simulink library "NxSwcLib"  (R2024a)
settings: Solver=VariableStepAuto  StartTime=0.0  StopTime=10.0  RelTol=1e-3
undefined symbols (not defined in the file or in its folder): QLF_DEBOUNCE, QLF_ERROR_RANGE, QLF_OK
libraries: simulink x4
Description:
  | SPDX-License-Identifier: Apache-2.0. neXtBSW block library for software components (RTE-07), generated by tools/swc/swc_lib_create.m - do not edit by hand.
settings Model: Creator=danie  LastModifiedBy=danie

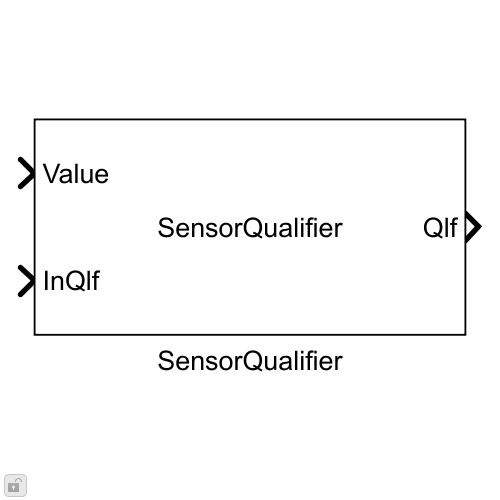
[thumbnail: Simulink's stored preview of the top-level diagram]
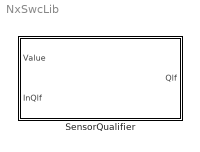
== system NxSwcLib ==
  SensorQualifier : Subsystem  mask(neXtBSW Sensor Qualifier){min_value=0, max_value=4095, debounce_ms=0}
      mask prompts: min_value "Lowest valid value (inclusive, unit of Value)"; max_value "Highest valid value (inclusive, unit of Value)"; debounce_ms "Debounce time of a range violation [ms] (0 = at once)"
      mask help:
      | Signal qualifier of a measured value (RTE-07). One value with precedence:
      | 1. InQlf ~= QLF_OK: InQlf unchanged (source not valid)
      | 2. Value outside [min_value, max_value] for at least debounce_ms: QLF_ERROR_RANGE
      | 3. Value outside, debounce time running: QLF_DEBOUNCE
      | 4. otherwise QLF_OK
      | The range is inclusive (NaN is not detected). The debounce time grows by the period of the calling runnable (sample time) from 0 at the first call outside the range; debounce_ms = 0 reports at once. Healing is immediate. Without a source qualifier connect a Constant QLF_OK to InQlf.
      mask init:
      | if ~isscalar(debounce_ms) || ~isreal(debounce_ms) || debounce_ms < 0 || debounce_ms ~= floor(debounce_ms) || debounce_ms > 2147483647
      |     error('SensorQualifier: debounce_ms must be a whole number of milliseconds from 0 to 2147483647');
      | end
      | if ~isscalar(min_value) || ~isscalar(max_value) || ~(min_value <= max_value)
      |     error('SensorQualifier: min_value must not be greater than max_value');
      | end
      mask Display:
      | disp('SensorQualifier');
      | port_label('input', 1, 'Value');
      | port_label('input', 2, 'InQlf');
      | port_label('output', 1, 'Qlf');

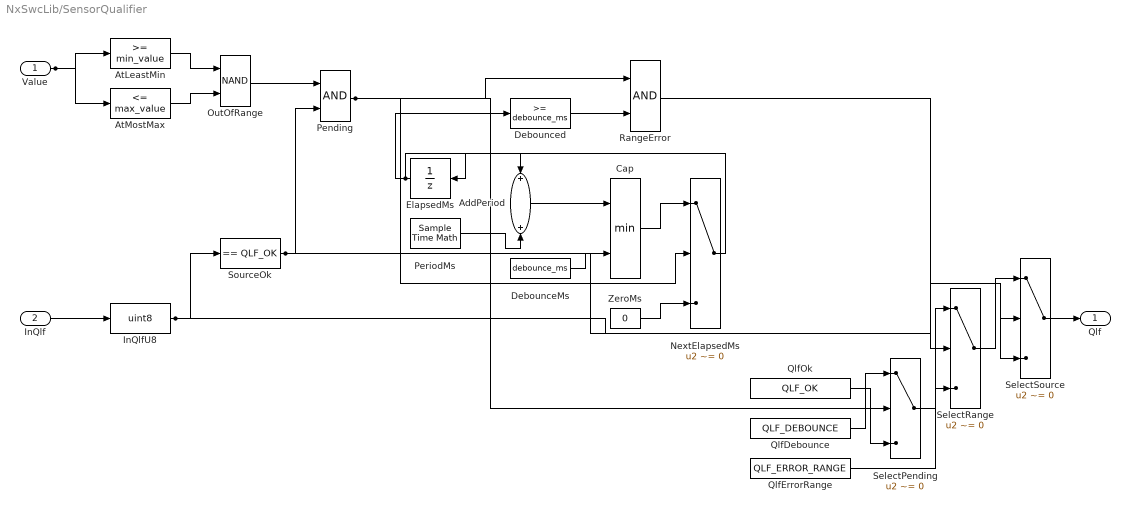
== system NxSwcLib/SensorQualifier ==
  Value : Inport
  InQlf : Inport  Port=2
  AddPeriod : Sum  OutDataTypeStr=uint32
  AtLeastMin : simulink/Logic and Bit Operations/Compare To Constant  relop=>=  const=min_value  OutDataTypeStr=boolean
  AtMostMax : simulink/Logic and Bit Operations/Compare To Constant  relop=<=  const=max_value  OutDataTypeStr=boolean
  Cap : MinMax  Inputs=2
  DebounceMs : Constant  Value=debounce_ms  OutDataTypeStr=uint32
  Debounced : simulink/Logic and Bit Operations/Compare To Constant  relop=>=  const=debounce_ms  OutDataTypeStr=boolean
  ElapsedMs : UnitDelay  SampleTime=-1  HasFrameUpgradeWarning=on
  InQlfU8 : DataTypeConversion  OutDataTypeStr=uint8  RndMeth=Floor
  NextElapsedMs : Switch  Criteria=u2 ~= 0  SaturateOnIntegerOverflow=off  InputSameDT=off
  OutOfRange : Logic  Operator=NAND  AllPortsSameDT=off  OutDataTypeStr=boolean
  Pending : Logic  AllPortsSameDT=off  OutDataTypeStr=boolean
  PeriodMs : SampleTimeMath  TsampMathOp=Ts Only  weightValue=1000  OutDataTypeStr=uint32  RndMeth=Nearest
  QlfDebounce : Constant  Value=QLF_DEBOUNCE  OutDataTypeStr=uint8
  QlfErrorRange : Constant  Value=QLF_ERROR_RANGE  OutDataTypeStr=uint8
  QlfOk : Constant  Value=QLF_OK  OutDataTypeStr=uint8
  RangeError : Logic  AllPortsSameDT=off  OutDataTypeStr=boolean
  SelectPending : Switch  Criteria=u2 ~= 0  SaturateOnIntegerOverflow=off  InputSameDT=off
  SelectRange : Switch  Criteria=u2 ~= 0  SaturateOnIntegerOverflow=off  InputSameDT=off
  SelectSource : Switch  Criteria=u2 ~= 0  SaturateOnIntegerOverflow=off  InputSameDT=off
  SourceOk : simulink/Logic and Bit Operations/Compare To Constant  relop===  const=QLF_OK  OutDataTypeStr=boolean
  ZeroMs : Constant  Value=0  OutDataTypeStr=uint32
  Qlf : Outport  OutDataTypeStr=uint8
  wires:
  Value/1 -> AtLeastMin/1, AtMostMax/1
  AtLeastMin/1 -> OutOfRange/1
  AtMostMax/1 -> OutOfRange/2
  InQlf/1 -> InQlfU8/1
  InQlfU8/1 -> SourceOk/1, SelectSource/3
  OutOfRange/1 -> Pending/1
  SourceOk/1 -> Pending/2, SelectSource/2
  ElapsedMs/1 -> AddPeriod/1, Debounced/1
  PeriodMs/1 -> AddPeriod/2
  AddPeriod/1 -> Cap/1
  DebounceMs/1 -> Cap/2
  Cap/1 -> NextElapsedMs/1
  Pending/1 -> NextElapsedMs/2, RangeError/1, SelectPending/2
  ZeroMs/1 -> NextElapsedMs/3
  NextElapsedMs/1 -> ElapsedMs/1
  Debounced/1 -> RangeError/2
  QlfDebounce/1 -> SelectPending/1
  QlfOk/1 -> SelectPending/3
  QlfErrorRange/1 -> SelectRange/1
  RangeError/1 -> SelectRange/2
  SelectPending/1 -> SelectRange/3
  SelectRange/1 -> SelectSource/1
  SelectSource/1 -> Qlf/1
